simulink model "DT_WNOPP_Twin"  (R2025b)
settings: Solver=FixedStepDiscrete  StartTime=0  StopTime=141  FixedStep=1  RelTol=1e-3
settings Model: Creator=HP  LastModifiedBy=HP

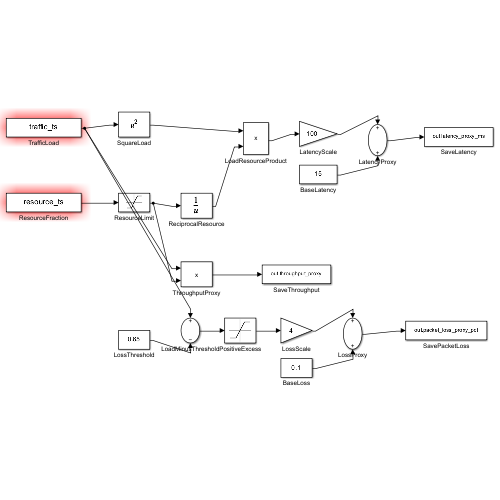
[thumbnail: Simulink's stored preview of the top-level diagram]
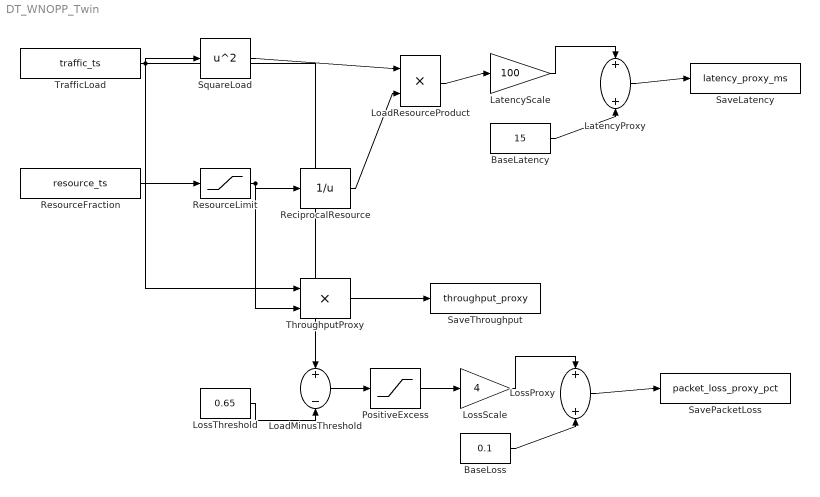
== system DT_WNOPP_Twin ==
  BaseLatency : Constant  Value=15
  BaseLoss : Constant  Value=0.1
  LatencyProxy : Sum
  LatencyScale : Gain  Gain=100
  LoadMinusThreshold : Sum  Inputs=+-
  LoadResourceProduct : Product
  LossProxy : Sum
  LossScale : Gain  Gain=4
  LossThreshold : Constant  Value=0.65
  PositiveExcess : Saturate  UpperLimit=1  LowerLimit=0
  ReciprocalResource : Math  Operator=reciprocal
  ResourceFraction : FromWorkspace  VariableName=resource_ts
  ResourceLimit : Saturate  UpperLimit=1  LowerLimit=0.1
  SaveLatency : ToWorkspace  VariableName=latency_proxy_ms  SaveFormat=Timeseries  SampleTime=-1
  SavePacketLoss : ToWorkspace  VariableName=packet_loss_proxy_pct  SaveFormat=Timeseries  SampleTime=-1
  SaveThroughput : ToWorkspace  VariableName=throughput_proxy  SaveFormat=Timeseries  SampleTime=-1
  SquareLoad : Math  Operator=square
  ThroughputProxy : Product
  TrafficLoad : FromWorkspace  VariableName=traffic_ts
  wires:
  TrafficLoad/1 -> SquareLoad/1, ThroughputProxy/1, LoadMinusThreshold/1
  ResourceFraction/1 -> ResourceLimit/1
  ResourceLimit/1 -> ReciprocalResource/1, ThroughputProxy/2
  SquareLoad/1 -> LoadResourceProduct/1
  ReciprocalResource/1 -> LoadResourceProduct/2
  LoadResourceProduct/1 -> LatencyScale/1
  LatencyScale/1 -> LatencyProxy/1
  BaseLatency/1 -> LatencyProxy/2
  LatencyProxy/1 -> SaveLatency/1
  ThroughputProxy/1 -> SaveThroughput/1
  LossThreshold/1 -> LoadMinusThreshold/2
  LoadMinusThreshold/1 -> PositiveExcess/1
  PositiveExcess/1 -> LossScale/1
  LossScale/1 -> LossProxy/1
  BaseLoss/1 -> LossProxy/2
  LossProxy/1 -> SavePacketLoss/1
